simulink model "force_position_step2_Vint"  (R2025b)
settings: Solver=VariableStepAuto  StartTime=0.0  StopTime=1  RelTol=1e-3
values from neighbouring files (symbols this model uses):
  lut_i_mA = interp1(z_anchor_um, i_anchor_mA, lut_z_um, 'pchip')    [init_force_position_sim_step2.m]
  lut_z_um = linspace(min(z_anchor_um), max(z_anchor_um), 501)    [init_force_position_sim_step2.m]
settings Model: Creator=HYB  LastModifiedBy=HYB

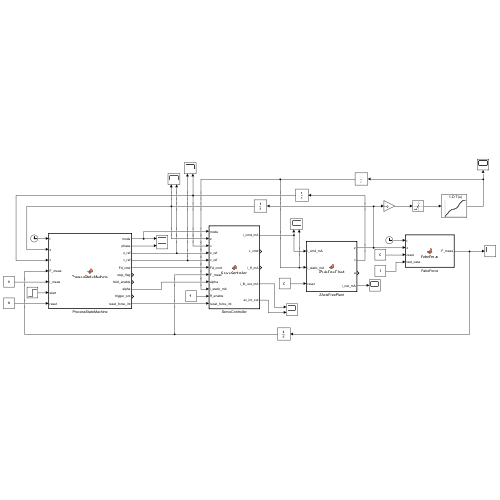
[thumbnail: Simulink's stored preview of the top-level diagram]
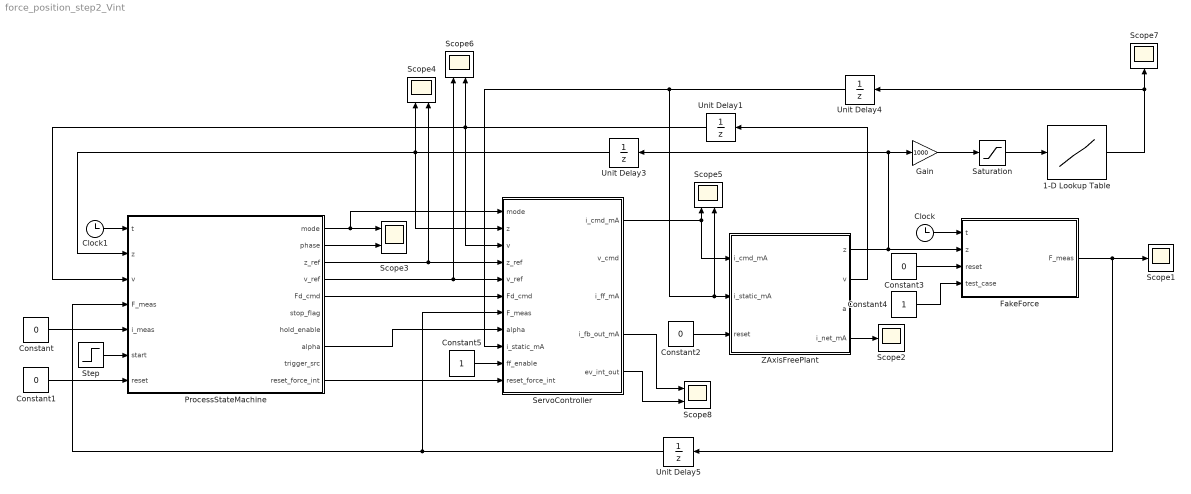
== system force_position_step2_Vint ==
  1-D Lookup Table : Lookup_n-D  NumberOfTableDimensions=1  BreakpointsForDimension1=lut_z_um  Table=lut_i_mA  InternalRulePriority=Speed  RndMeth=Simplest
  Clock : Clock
  Clock1 : Clock
  Constant{,1..3} (4 alike) : Constant  Value=0
  Constant4 : Constant
  Constant5 : Constant
  FakeForce : MATLAB Function  TreatAsAtomicUnit=on
  Gain : Gain  Gain=1000
  ProcessStateMachine : MATLAB Function  TreatAsAtomicUnit=on
  Saturation : Saturate  UpperLimit=15000  LowerLimit=0
  Scope1 : Scope
      settings: ActiveDisplayYMinimum=-2.4999999999999996  ActiveDisplayYMaximum=22.5
  Scope2 : Scope
      settings: ActiveDisplayYMinimum=-1967.6933461484089  ActiveDisplayYMaximum=1895.5357153815362
  Scope{3..6,8} (5 alike) : Scope  NumInputPorts=2
      Scope3 settings: ActiveDisplayYMinimum=-0.49999999999999989  ActiveDisplayYMaximum=4.5  DataLoggingVariableName=ScopeData3
      Scope4 settings: ActiveDisplayYMinimum=12.384517457906124  ActiveDisplayYMaximum=15.319237234661129  DataLoggingVariableName=ScopeData4
      Scope5 settings: ActiveDisplayYMinimum=-403.88890728908666  ActiveDisplayYMaximum=1479.7302904427656  DataLoggingVariableName=ScopeData5
      Scope6 settings: ActiveDisplayYMinimum=-286.20412971277597  ActiveDisplayYMaximum=250.96623524657483  DataLoggingVariableName=ScopeData6
      Scope8 settings: ActiveDisplayYMinimum=-0.74701256142848438  ActiveDisplayYMaximum=0.76648242555809953  DataLoggingVariableName=ScopeData2
  Scope7 : Scope
      settings: ActiveDisplayYMinimum=645.6688347730925  ActiveDisplayYMaximum=873.33389076398271  DataLoggingVariableName=ScopeData7
  ServoController : MATLAB Function  TreatAsAtomicUnit=on
  Step : Step  Time=0.01  SampleTime=0
  Unit Delay{1,3..5} (4 alike) : UnitDelay  SampleTime=0.001  HasFrameUpgradeWarning=on
  ZAxisFreePlant : MATLAB Function  TreatAsAtomicUnit=on
  wires:
  ProcessStateMachine/1(mode) -> Scope3/1, ServoController/1(mode)
  ProcessStateMachine/10(reset_force_int) -> ServoController/11(reset_force_int)
  Unit Delay3/1 -> ProcessStateMachine/2(z), Scope4/1, ServoController/2(z)
  Step/1 -> ProcessStateMachine/6(start)
  1-D Lookup Table/1 -> Unit Delay4/1, Scope7/1
  Constant2/1 -> ZAxisFreePlant/3(reset)
  ZAxisFreePlant/4(i_net_mA) -> Scope2/1
  ProcessStateMachine/8(alpha) -> ServoController/8(alpha)
  ProcessStateMachine/3(z_ref) -> Scope4/2, ServoController/4(z_ref)
  ZAxisFreePlant/1(z) -> FakeForce/2(z), Unit Delay3/1, Gain/1
  Unit Delay4/1 -> Scope5/2, ZAxisFreePlant/2(i_static_mA), ServoController/9(i_static_mA)
  Gain/1 -> Saturation/1
  Constant/1 -> ProcessStateMachine/5(i_meas)
  ProcessStateMachine/4(v_ref) -> ServoController/5(v_ref), Scope6/1
  ProcessStateMachine/5(Fd_cmd) -> ServoController/6(Fd_cmd)
  Constant1/1 -> ProcessStateMachine/7(reset)
  Clock1/1 -> ProcessStateMachine/1(t)
  Unit Delay5/1 -> ProcessStateMachine/4(F_meas), ServoController/7(F_meas)
  ZAxisFreePlant/2(v) -> Unit Delay1/1
  ProcessStateMachine/2(phase) -> Scope3/2
  Constant4/1 -> FakeForce/4(test_case)
  Constant5/1 -> ServoController/10(ff_enable)
  ServoController/1(i_cmd_mA) -> ZAxisFreePlant/1(i_cmd_mA), Scope5/1
  Saturation/1 -> 1-D Lookup Table/1
  Unit Delay1/1 -> ServoController/3(v), ProcessStateMachine/3(v), Scope6/2
  ServoController/4(i_fb_out_mA) -> Scope8/1
  ServoController/5(ev_int_out) -> Scope8/2
  Clock/1 -> FakeForce/1(t)
  Constant3/1 -> FakeForce/3(reset)
  FakeForce/1(F_meas) -> Unit Delay5/1, Scope1/1

== matlab function force_position_step2_Vint/ZAxisFreePlant ==
  data: i_cmd_mA input; z output; i_static_mA input; reset input; v output; a output; i_net_mA output
function [z, v, a, i_net_mA] = ZAxisFreePlant(i_cmd_mA, i_static_mA, reset)
%#codegen

% ============================================================
% 简化Z轴自由运动模型
%
% 下行方向为正：
%   z 增大表示压头向下伸出
%
% i_static_mA 是实验一得到的下行静态保持电流。
% 在对象模型中，它作为位置相关的非线性负载项。
%
% 简化模型：
%   a = Kacc * (i_cmd - i_static(z) - Cv*v - Icoul*tanh(v/vs))
% ============================================================

%% 参数
Ts = 1e-3;

z0 = 0.0;          % 初始位置，mm
v0 = 0.0;

z_min = 0.0;
z_max = 15.2;      % 比实际15mm略大一点，便于保护观察

Kacc = 20.0;        % mm/s^2 per mA
Cv_mA = 1.0;       % mA/(mm/s)
Icoul_mA = 2.0;    % mA
vs = 0.05;         % mm/s，tanh平滑速度

persistent z_k v_k

if isempty(z_k)
    z_k = z0;
    v_k = v0;
end

if reset
    z_k = z0;
    v_k = v0;
end

%% 摩擦电流，平滑符号函数
i_fric_mA = Cv_mA * v_k + Icoul_mA * tanh(v_k / vs);

%% 净驱动电流
i_net_mA = i_cmd_mA - i_static_mA - i_fric_mA;

%% 加速度
a = Kacc * i_net_mA;

%% 积分
v_k = v_k + Ts * a;
z_k = z_k + Ts * v_k;

%% 行程限位
if z_k < z_min
    z_k = z_min;
    if v_k < 0
        v_k = 0.0;
    end
elseif z_k > z_max
    z_k = z_max;
    if v_k > 0
        v_k = 0.0;
    end
end

z = z_k;
v = v_k;

== matlab function force_position_step2_Vint/ServoController ==
  data: mode input; i_cmd_mA output; z input; v input; z_ref input; v_ref input; Fd_cmd input; F_meas input; alpha input; i_static_mA input; ff_enable input; reset_force_int input; v_cmd output; i_ff_mA output; i_fb_out_mA output; ev_int_out output
function [i_cmd_mA, v_cmd, i_ff_mA, i_fb_out_mA, ev_int_out] = ServoController( ...
    mode, z, v, z_ref, v_ref, Fd_cmd, F_meas, alpha, ...
    i_static_mA, ff_enable, reset_force_int)
%#codegen

% ============================================================
% 简化伺服控制器：位置外环 + 速度PI内环 + 静态前馈
%
% mode = 1: 位置模式
% mode = 2: 速度模式
% mode = 3: 保压/力矩模式，第二步暂时用速度为0的保持逻辑
% mode = 9: 安全停止
%
% 主要修改：
% 1. 速度环由 P 改为 PI；
% 2. 无静态前馈时，积分项可以补偿静态负载；
% 3. 有静态前馈时，积分负担明显减小。
% ============================================================

%% 基本参数
Ts = 1e-3;

%% 位置环参数
Kp_pos = 100.0;       % 位置环比例，输出速度
v_fast_max = 100.0;   % 位置模式最大速度，mm/s

%% 速度PI参数
Kvp = 20.0;           % 速度比例增益，mA/(mm/s)
Kvi = 200.0;          % 速度积分增益，mA/mm

i_limit = 5000.0;     % 电流限幅，mA
i_int_limit = 3000.0; % 积分项限幅，mA

%% 力控参数，第三步再正式使用
Kforce = 1.0;
Kpf = 0.0;
Kif = 0.0;

persistent ev_int eF_int last_mode

if isempty(ev_int)
    ev_int = 0.0;
    eF_int = 0.0;
    last_mode = 0.0;
end

%% 如果复位，则清空积分
if reset_force_int
    eF_int = 0.0;
end

%% 模式切换时，可以适当清理速度积分
% 注意：这里不建议每次从位置到速度都清零，否则积分刚建立又被清掉。
% 只在进入错误停止或重新开始时清空。
if mode == 9
    ev_int = 0.0;
end

%% 默认量
v_cmd = 0.0;
i_force_ff_mA = 0.0;
i_force_fb_mA = 0.0;

%% 生成速度指令
if mode == 1
    % 位置模式：位置误差生成速度指令
    e_pos = z_ref - z;
    v_cmd = Kp_pos * e_pos;
    
    if v_cmd > v_fast_max
        v_cmd = v_fast_max;
    elseif v_cmd < -v_fast_max
        v_cmd = -v_fast_max;
    end

elseif mode == 2
    % 速度模式
    v_cmd = v_ref;

elseif mode == 3
    % 第二步暂时不接触真实环境，进入保压后先保持速度为0
    v_cmd = 0.0;

elseif mode == 9
    v_cmd = 0.0;

else
    v_cmd = 0.0;
end

%% 速度PI控制
if mode == 1 || mode == 2 || mode == 3
    e_v = v_cmd - v;
    
    % 先计算未积分前的比例项
    i_p = Kvp * e_v;
    
    % 积分更新
    ev_int = ev_int + e_v * Ts;
    
    % 积分项限幅，防止积分过大
    i_i = Kvi * ev_int;
    
    if i_i > i_int_limit
        i_i = i_int_limit;
        ev_int = i_i / Kvi;
    elseif i_i < -i_int_limit
        i_i = -i_int_limit;
        ev_int = i_i / Kvi;
    end
    
    i_fb_mA = i_p + i_i;
else
    e_v = 0.0;
    i_fb_mA = 0.0;
end

%% 静态前馈
if ff_enable > 0.5
    i_ff_mA = i_static_mA;
else
    i_ff_mA = 0.0;
end

%% 后续力前馈和力反馈，第二步暂时不启用
if mode == 3
    % 后续第三步可启用：
    % i_force_ff_mA = alpha * Kforce * Fd_cmd;
    % eF = Fd_cmd - F_meas;
    % eF_int = eF_int + eF * Ts;
    % i_force_fb_mA = Kpf * eF + Kif * eF_int;
    i_force_ff_mA = 0.0;
    i_force_fb_mA = 0.0;
end

%% 合成电流
i_cmd_unsat = i_ff_mA + i_fb_mA + i_force_ff_mA + i_force_fb_mA;

%% 总电流限幅
i_cmd_mA = i_cmd_unsat;

if i_cmd_mA > i_limit
    i_cmd_mA = i_limit;
elseif i_cmd_mA < -i_limit
    i_cmd_mA = -i_limit;
end

%% 简单抗饱和处理
% 如果总输出饱和，并且积分还在推动饱和方向，则减缓积分增长
if i_cmd_unsat ~= i_cmd_mA
    if (i_cmd_unsat > i_limit && e_v > 0) || (i_cmd_unsat < -i_limit && e_v < 0)
        ev_int = ev_int - 0.5 * e_v * Ts;
    end
end

%% 输出观测量
i_fb_out_mA = i_fb_mA;
ev_int_out = ev_int;

last_mode = mode;

== matlab function force_position_step2_Vint/ProcessStateMachine ==
  data: t input; mode output; z input; v input; F_meas input; i_meas input; start input; reset input; phase output; z_ref output; v_ref output; Fd_cmd output; stop_flag output; hold_enable output; alpha output; trigger_src output; reset_force_int output
function [mode, phase, z_ref, v_ref, Fd_cmd, stop_flag, hold_enable, alpha, trigger_src, reset_force_int] = ...
    ProcessStateMachine(t, z, v, F_meas, i_meas, start, reset)
%#codegen

% ============================================================
% 力位控制工艺流程状态机
% 阶段：
% 0 Ready
% 1 FastPosition: 位置模式快进到 13 mm
% 2 FirstVelocity: 第一速度到 14 mm
% 3 SearchVelocity: 第二速度搜索接触
% 4 ForceHold: 力矩/电流模式保压
% 5 ErrorStop: 超行程或异常停止
% ============================================================


%% ---------- 可调参数 ----------
z_fast_end = 13.0;     % mm
z_v1_end   = 14.0;     % mm
z_max      = 15.0;     % mm

pos_tol = 0.02;        % mm

v1_search = 10.0;       % mm/s
v2_search = 0.2;       % mm/s

F_th = 5.0;           % g
T_force_confirm = 0.001;   % s

v_stop_th = 0.05;          % mm/s
T_v_confirm = 0.005;       % s

% 第一版暂不启用电流判断，所以阈值给很大
i_stop_th = 1e9;
T_i_confirm = 0.003;       % s

Fd_set = 200.0;            % g
T_ramp_force = 0.010;      % s

%% ---------- 状态变量 ----------
persistent state t_enter tF_start tV_start tI_start prev_state

if isempty(state)
    state = int32(0);
    prev_state = int32(0);
    t_enter = 0.0;
    tF_start = -1.0;
    tV_start = -1.0;
    tI_start = -1.0;
end

if reset
    state = int32(0);
    prev_state = int32(0);
    t_enter = t;
    tF_start = -1.0;
    tV_start = -1.0;
    tI_start = -1.0;
end

%% ---------- 默认输出 ----------
mode = 0;
phase = double(state);
z_ref = z; % 默认保持住位置，防止突然运动
v_ref = 0.0;
Fd_cmd = Fd_set; % 默认力指令就设置为力设定值，切换为力控时目标力则已经是设定值
stop_flag = false; % 默认不停止，运行外部控制器继续执行位置/速度环
hold_enable = false; % 默认禁用积分器保持，在状态4会开启，力控时造成的位移累积误差在切换回位控时可以快速恢复
alpha = 0.0; % 在状态4时会从0平滑过渡到1
trigger_src = 0;       % 0 none, 1 force, 2 velocity, 3 current, 4 z_max
reset_force_int = false; % 默认不复位力控积分器，只在进入状态4的瞬间设1

prev_state = state;

%% ---------- 启动逻辑 ----------
if state == 0
    mode = 0;
    phase = 0;
    z_ref = z;
    v_ref = 0.0;
    alpha = 0.0;
    
    if start % 一般阶跃输入
        state = int32(1);
        t_enter = t; % 进入当前状态的时间戳
    end
end

%% ---------- 状态 1：位置快进 ----------
if state == 1
    mode = 1;
    phase = 1;
    z_ref = z_fast_end;
    v_ref = 0.0;
    alpha = 0.0;
    
    if z >= z_fast_end - pos_tol
        state = int32(2);
        t_enter = t;
    end
end

%% ---------- 状态 2：第一速度 ----------
if state == 2
    mode = 2;          % 速度模式
    phase = 2;
    z_ref = z;
    v_ref = v1_search;
    alpha = 0.0;
    
    if z >= z_v1_end - pos_tol
        state = int32(3);
        t_enter = t;
        tF_start = -1.0;
        tV_start = -1.0;
        tI_start = -1.0;
    end
end

%% ---------- 状态 3：第二速度搜索 ----------
if state == 3
    mode = 2;          % 速度模式
    phase = 3;
    z_ref = z;
    v_ref = v2_search;
    alpha = 0.0;
    
    % --- 压力触发 ---
    if F_meas > F_th
        if tF_start < 0.0
            tF_start = t;
        end
    else
        tF_start = -1.0;
    end
    
    force_ok = false;
    if tF_start >= 0.0
        if (t - tF_start) >= T_force_confirm
            force_ok = true;
        end
    end
    
    % --- 速度触发，第一版作为备用 ---
    if abs(v) < v_stop_th
        if tV_start < 0.0
            tV_start = t;
        end
    else
        tV_start = -1.0;
    end
    
    velocity_ok = false;
    if tV_start >= 0.0
        if (t - tV_start) >= T_v_confirm
            velocity_ok = true;
        end
    end
    
    % --- 电流触发，第一版实际不会触发 ---
    if abs(i_meas) > i_stop_th
        if tI_start < 0.0
            tI_start = t;
        end
    else
        tI_start = -1.0;
    end
    
    current_ok = false;
    if tI_start >= 0.0
        if (t - tI_start) >= T_i_confirm
            current_ok = true;
        end
    end
    
    % --- 停止条件 ---
    if force_ok
        state = int32(4);
        t_enter = t;
        trigger_src = 1;
        stop_flag = true;
    elseif velocity_ok
        state = int32(4);
        t_enter = t;
        trigger_src = 2;
        stop_flag = true;
    elseif current_ok
        state = int32(4);
        t_enter = t;
        trigger_src = 3;
        stop_flag = true;
    elseif z >= z_max
        state = int32(5);
        t_enter = t;
        trigger_src = 4;
    end
end

%% ---------- 状态 4：力矩/电流模式保压 ----------
if state == 4
    mode = 3;          % 力矩/电流模式
    phase = 4;
    z_ref = z;
    v_ref = 0.0;
    Fd_cmd = Fd_set;
    stop_flag = true;
    hold_enable = true;
    
    % 目标力前馈平滑引入系数 alpha: 0 -> 1
    tau = (t - t_enter) / T_ramp_force;
    if tau < 0.0
        tau = 0.0;
    elseif tau > 1.0
        tau = 1.0;
    end
    
    % S型平滑
    alpha = 3.0*tau*tau - 2.0*tau*tau*tau;
end

%% ---------- 状态 5：安全停止 ----------
if state == 5
    mode = 9;
    phase = 5;
    z_ref = z;
    v_ref = 0.0;
    Fd_cmd = 0.0;
    stop_flag = true;
    hold_enable = false;
    alpha = 0.0;
end

%% ---------- 进入保压瞬间复位力控积分 ----------
if prev_state ~= int32(4) && state == int32(4)
    reset_force_int = true;
else
    reset_force_int = false;
end

phase = double(state);

== matlab function force_position_step2_Vint/FakeForce ==
  data: t input; z input; F_meas output; reset input; test_case input
function F_meas = FakeForce(t, z, reset, test_case)
%#codegen

% ============================================================
% 假力信号发生器，仅用于状态机测试
%
% test_case = 1：正常接触，z >= 14.5 mm 后持续产生力
% test_case = 2：始终无接触，测试最大行程保护
% test_case = 3：短暂误触发，测试持续时间确认逻辑
% test_case = 4：不产生力，配合 IdealAxisPlant 测试速度停止触发
% ============================================================

z_contact = 14.3;      % mm
F_contact = 20.0;      % g

persistent t_cross crossed

if isempty(t_cross)
    t_cross = -1.0;
    crossed = false;
end

if reset
    t_cross = -1.0;
    crossed = false;
end

F_meas = 0.0;

if test_case == 1
    % 正常接触：到达 14.5 mm 后持续有力
    if z >= z_contact
        F_meas = F_contact;
    else
        F_meas = 0.0;
    end
    
elseif test_case == 2
    % 无接触：始终为 0
    F_meas = 0.0;
    
elseif test_case == 3
    % 短暂误触发：只给 1 ms 左右的力脉冲
    if z >= z_contact && ~crossed
        crossed = true;
        t_cross = t;
    end
    
    if crossed
        if (t - t_cross) <= 0.001
            F_meas = F_contact;
        else
            F_meas = 0.0;
        end
    end
    
elseif test_case == 4
    % 不产生力，用于测试速度触发条件
    F_meas = 0.0;
    
else
    F_meas = 0.0;
end
